simulink model "case_05_slow_to_fast_mid_transition"  (R2025b)
settings: Solver=VariableStepAuto  StartTime=0.0  StopTime=30  RelTol=1e-3
settings Model: Creator=sanborkl  LastModifiedBy=sanborkl

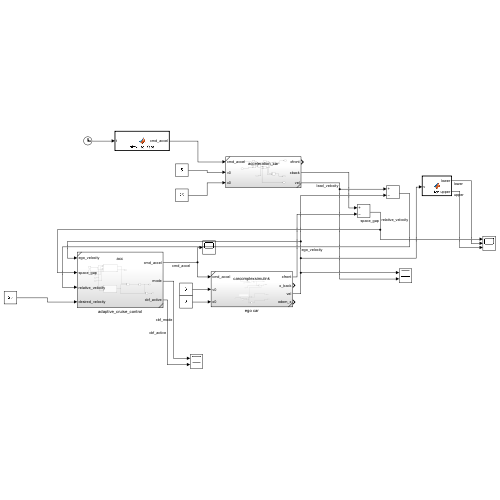
[thumbnail: Simulink's stored preview of the top-level diagram]
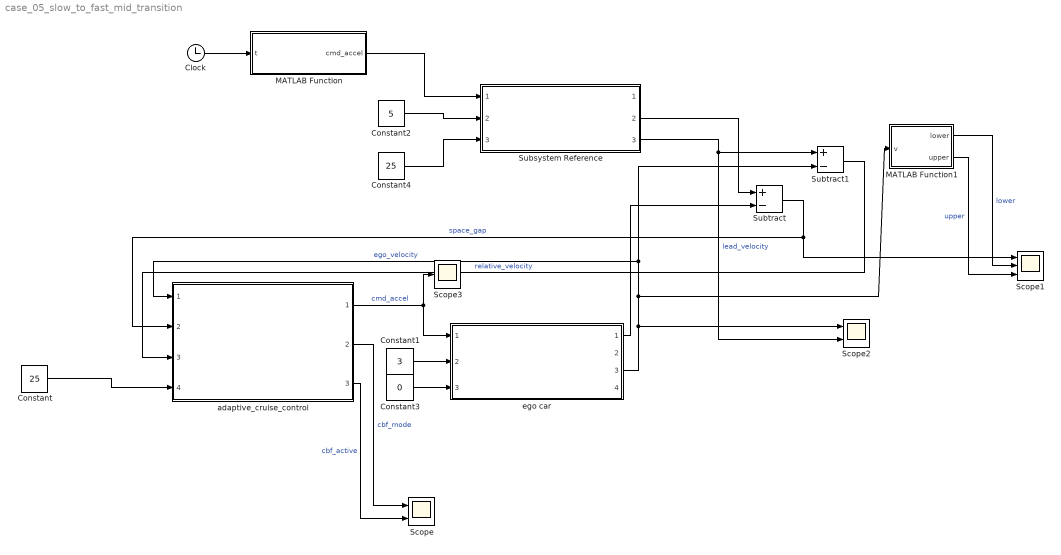
== system case_05_slow_to_fast_mid_transition ==
  Clock : Clock
  Constant : Constant  Value=25
  Constant1 : Constant  Value=3
  Constant2 : Constant  Value=5
  Constant3 : Constant  Value=0
  Constant4 : Constant  Value=25
  MATLAB Function : MATLAB Function  TreatAsAtomicUnit=on
  MATLAB Function1 : MATLAB Function  TreatAsAtomicUnit=on
  Scope : Scope  NumInputPorts=2
      settings: ActiveDisplayYMinimum=0.9  ActiveDisplayYMaximum=1.1
  Scope1 : Scope  NumInputPorts=3
      settings: ActiveDisplayYMinimum=4.1752293602675881  ActiveDisplayYMaximum=72.422935757591716  YLabel=m
  Scope2 : Scope  NumInputPorts=2
      settings: ActiveDisplayYMinimum=-0.025792650607180168  ActiveDisplayYMaximum=30.232133855464628  YLabel=m/s  DataLoggingVariableName=ScopeData2
  Scope3 : Scope
      settings: ActiveDisplayYMinimum=-1.9080470211396121  ActiveDisplayYMaximum=1.5724231902565085  YLabel=m/s^2  DataLoggingVariableName=ScopeData3
  Subsystem Reference : Subsystem  ReferencedSubsystem=acceleration_car
  Subtract : Sum  Inputs=+-
  Subtract1 : Sum  Inputs=+-
  adaptive_cruise_control : Subsystem  ReferencedSubsystem=acc
  ego car : Subsystem  ReferencedSubsystem=carcomplexsimulink
  wires:
  ego car/3 -> Subtract1/2, adaptive_cruise_control/1, MATLAB Function1/1(v), Scope2/1  "ego_velocity"
  adaptive_cruise_control/1 -> ego car/1, Scope3/1  "cmd_accel"
  Constant1/1 -> ego car/2
  Subtract1/1 -> adaptive_cruise_control/3  "relative_velocity"
  Subsystem Reference/3 -> Scope2/2, Subtract1/1  "lead_velocity"
  Constant3/1 -> ego car/3
  MATLAB Function/1(cmd_accel) -> Subsystem Reference/1
  Constant2/1 -> Subsystem Reference/2
  adaptive_cruise_control/2 -> Scope/1  "cbf_mode"
  Subsystem Reference/2 -> Subtract/1
  adaptive_cruise_control/3 -> Scope/2  "cbf_active"
  Constant/1 -> adaptive_cruise_control/4
  ego car/1 -> Subtract/2
  Subtract/1 -> Scope1/1, adaptive_cruise_control/2  "space_gap"
  Constant4/1 -> Subsystem Reference/3
  Clock/1 -> MATLAB Function/1(t)
  MATLAB Function1/1(lower) -> Scope1/2  "lower"
  MATLAB Function1/2(upper) -> Scope1/3  "upper"

== matlab function case_05_slow_to_fast_mid_transition/MATLAB Function ==
  data: t input; cmd_accel output
function cmd_accel = slow_to_fast(t)

if t < 1
    cmd_accel = sin(t);
else
    cmd_accel = 0.75;
end

== matlab function case_05_slow_to_fast_mid_transition/MATLAB Function1 ==
  data: v input; lower output; upper output
function [lower, upper] = fcn(v)

lower = 2 * v + 5;
upper = 2 * v + 15;
